simulink model "cable_driven_parallel_robot2022"  (R2022b)
settings: Solver=ode3  StartTime=0.0  StopTime=100  FixedStep=0.01  RelTol=1e-3
values from neighbouring files (symbols this model uses):
  cable_length = 1.2    [Model_Info.m]
  g = 9.81    [Model_Info.m]
  MP_H = 2    [Model_Info.m]
  MP_init_X = 0    [Model_Info.m]
  MP_init_Y = 0    [Model_Info.m]
  MP_init_Z = cable_length + (MP_H/2)    (= 2.2)    [Model_Info.m]
  MP_Ix = (MP_m/12)*(MP_W^2+MP_H^2)    (= 6.66666666667e-05)    [Model_Info.m]
  MP_Iy = (MP_m/12)*(MP_L^2+MP_H^2)    (= 6.66666666667e-05)    [Model_Info.m]
  MP_Iz = (MP_m/12)*(MP_L^2+MP_W^2)    (= 6.66666666667e-05)    [Model_Info.m]
  MP_L = 2    [Model_Info.m]
  MP_m = 0.0001    [Model_Info.m]
  MP_W = 2    [Model_Info.m]
  MR_init_X_L1 = -(MP_L/2)    (= -1)    [Model_Info.m]
  MR_init_X_L2 = (MP_L/2)    (= 1)    [Model_Info.m]
  MR_init_X_L3 = (MP_L/2)    (= 1)    [Model_Info.m]
  MR_init_X_L4 = -(MP_L/2)    (= -1)    [Model_Info.m]
  MR_init_Y_L1 = -(MP_W/2)    (= -1)    [Model_Info.m]
  MR_init_Y_L2 = -(MP_W/2)    (= -1)    [Model_Info.m]
  MR_init_Y_L3 = (MP_W/2)    (= 1)    [Model_Info.m]
  MR_init_Y_L4 = (MP_W/2)    (= 1)    [Model_Info.m]
  MR_init_Yaw_L1 = pi    (= 3.14159265359)    [Model_Info.m]
  MR_init_Yaw_L2 = 0    [Model_Info.m]
  MR_init_Yaw_L3 = 0    [Model_Info.m]
  MR_init_Yaw_L4 = pi    (= 3.14159265359)    [Model_Info.m]
  MR_Jr = (MR_m/12)*(MR_L^2+MR_W^2)    (= 0.333333333333)    [Model_Info.m]
  MR_m = 0.5    [Model_Info.m]
  MR_r = 2    [Model_Info.m]
  MR_WT = 2    [Model_Info.m]
  QR_Ax = 0.25*0    (= 0)    [Model_Info.m]
  QR_Ay = 0.25*0    (= 0)    [Model_Info.m]
  QR_Az = 0.25*0    (= 0)    [Model_Info.m]
  QR_b = 1.14*1e-7    (= 1.14e-07)    [Model_Info.m]
  QR_Ixx = 4.856*1e-3    (= 0.004856)    [Model_Info.m]
  QR_Iyy = 4.856*1e-3    (= 0.004856)    [Model_Info.m]
  QR_Izz = 8.801*1e-3    (= 0.008801)    [Model_Info.m]
  QR_K = 2.980*1e-6    (= 2.98e-06)    [Model_Info.m]
  QR_l = 0.225    [Model_Info.m]
  QR_m = 0.468    [Model_Info.m]
  QR_x0_U1 = -(MP_L/2)    (= -1)    [Model_Info.m]
  QR_x0_U2 = (MP_L/2)    (= 1)    [Model_Info.m]
  QR_x0_U3 = (MP_L/2)    (= 1)    [Model_Info.m]
  QR_x0_U4 = -(MP_L/2)    (= -1)    [Model_Info.m]
  QR_y0_U1 = -(MP_W/2)    (= -1)    [Model_Info.m]
  QR_y0_U2 = -(MP_W/2)    (= -1)    [Model_Info.m]
  QR_y0_U3 = (MP_W/2)    (= 1)    [Model_Info.m]
  QR_y0_U4 = (MP_W/2)    (= 1)    [Model_Info.m]
  QR_z0_U1 = 2*cable_length+(MP_H)    (= 4.4)    [Model_Info.m]
  QR_z0_U2 = 2*cable_length+(MP_H)    (= 4.4)    [Model_Info.m]
  QR_z0_U3 = 2*cable_length+(MP_H)    (= 4.4)    [Model_Info.m]
  QR_z0_U4 = 2*cable_length+(MP_H)    (= 4.4)    [Model_Info.m]
(part 5 of 12)

== system cable_driven_parallel_robot2022/Actuators-CableTension-MovingPlatform/QuadRotor1/Subsystem/Subsystem ==
  rest : Inport
  init : Inport  Port=2
  MATLAB Function : MATLAB Function  TreatAsAtomicUnit=on
  A_rest : Outport
  A_init : Outport  Port=2
  wires:
  MATLAB Function/2(init) -> A_init/1
  init/1 -> MATLAB Function/2(init0)
  MATLAB Function/1(rest) -> A_rest/1
  rest/1 -> MATLAB Function/1(rest0)

== system cable_driven_parallel_robot2022/Actuators-CableTension-MovingPlatform/QuadRotor1/Subsystem/Subsystem1 ==
  rest : Inport
  init : Inport  Port=2
  MATLAB Function : MATLAB Function  TreatAsAtomicUnit=on
  A_rest : Outport
  A_init : Outport  Port=2
  wires:
  MATLAB Function/2(init) -> A_init/1
  init/1 -> MATLAB Function/2(init0)
  MATLAB Function/1(rest) -> A_rest/1
  rest/1 -> MATLAB Function/1(rest0)

== system cable_driven_parallel_robot2022/Actuators-CableTension-MovingPlatform/QuadRotor1/Subsystem/Vel_Manager ==
  Demux : Demux  Outputs=3
  Demux1 : Demux  Outputs=8
  Terminator{,1..6} (7 alike) : Terminator
  Vx_min : Outport
  Vy_min : Outport  Port=2
  Vz_min : Outport  Port=3
  Reste : Outport  Port=4
  wires:
  Demux1/7 -> Terminator5/1
  Demux1/3 -> Terminator1/1
  [Vmin] -> Demux/1
  Demux1/8 -> Terminator6/1
  [isTension] -> Demux1/1
  Demux1/6 -> Terminator4/1
  Demux1/5 -> Terminator3/1
  Demux1/4 -> Terminator2/1
  Demux/1 -> Vx_min/1
  Demux/2 -> Vy_min/1
  Demux/3 -> Vz_min/1
  Demux1/2 -> Reste/1
  Demux1/1 -> Terminator/1

== system cable_driven_parallel_robot2022/Actuators-CableTension-MovingPlatform/QuadRotor2/Subsystem/Subsystem ==
  rest : Inport
  init : Inport  Port=2
  MATLAB Function : MATLAB Function  TreatAsAtomicUnit=on
  A_rest : Outport
  A_init : Outport  Port=2
  wires:
  rest/1 -> MATLAB Function/1(rest0)
  MATLAB Function/1(rest) -> A_rest/1
  init/1 -> MATLAB Function/2(init0)
  MATLAB Function/2(init) -> A_init/1

== system cable_driven_parallel_robot2022/Actuators-CableTension-MovingPlatform/QuadRotor2/Subsystem/Subsystem1 ==
  rest : Inport
  init : Inport  Port=2
  MATLAB Function : MATLAB Function  TreatAsAtomicUnit=on
  A_rest : Outport
  A_init : Outport  Port=2
  wires:
  rest/1 -> MATLAB Function/1(rest0)
  MATLAB Function/1(rest) -> A_rest/1
  init/1 -> MATLAB Function/2(init0)
  MATLAB Function/2(init) -> A_init/1

== system cable_driven_parallel_robot2022/Actuators-CableTension-MovingPlatform/QuadRotor2/Subsystem/Vel_Manager ==
  Demux : Demux  Outputs=3
  Demux1 : Demux  Outputs=8
  Terminator{,1..6} (7 alike) : Terminator
  Vx_min : Outport
  Vy_min : Outport  Port=2
  Vz_min : Outport  Port=3
  Reste : Outport  Port=4
  wires:
  Demux1/7 -> Terminator5/1
  [Vmin] -> Demux/1
  Demux1/8 -> Terminator6/1
  [isTension] -> Demux1/1
  Demux1/6 -> Terminator4/1
  Demux1/2 -> Terminator/1
  Demux1/5 -> Terminator3/1
  Demux1/4 -> Terminator2/1
  Demux/1 -> Vx_min/1
  Demux/2 -> Vy_min/1
  Demux/3 -> Vz_min/1
  Demux1/3 -> Reste/1
  Demux1/1 -> Terminator1/1

== system cable_driven_parallel_robot2022/Actuators-CableTension-MovingPlatform/QuadRotor3/Subsystem/Subsystem ==
  rest : Inport
  init : Inport  Port=2
  MATLAB Function : MATLAB Function  TreatAsAtomicUnit=on
  A_rest : Outport
  A_init : Outport  Port=2
  wires:
  MATLAB Function/2(init) -> A_init/1
  init/1 -> MATLAB Function/2(init0)
  MATLAB Function/1(rest) -> A_rest/1
  rest/1 -> MATLAB Function/1(rest0)

== system cable_driven_parallel_robot2022/Actuators-CableTension-MovingPlatform/QuadRotor3/Subsystem/Subsystem1 ==
  rest : Inport
  init : Inport  Port=2
  MATLAB Function : MATLAB Function  TreatAsAtomicUnit=on
  A_rest : Outport
  A_init : Outport  Port=2
  wires:
  MATLAB Function/2(init) -> A_init/1
  init/1 -> MATLAB Function/2(init0)
  MATLAB Function/1(rest) -> A_rest/1
  rest/1 -> MATLAB Function/1(rest0)

== system cable_driven_parallel_robot2022/Actuators-CableTension-MovingPlatform/QuadRotor3/Subsystem/Vel_Manager ==
  Demux : Demux  Outputs=3
  Demux1 : Demux  Outputs=8
  Terminator{,1..6} (7 alike) : Terminator
  Vx_min : Outport
  Vy_min : Outport  Port=2
  Vz_min : Outport  Port=3
  Reste : Outport  Port=4
  wires:
  Demux1/7 -> Terminator5/1
  Demux1/3 -> Terminator1/1
  [Vmin] -> Demux/1
  Demux1/8 -> Terminator6/1
  [isTension] -> Demux1/1
  Demux1/6 -> Terminator4/1
  Demux1/2 -> Terminator/1
  Demux1/5 -> Terminator3/1
  Demux/1 -> Vx_min/1
  Demux/2 -> Vy_min/1
  Demux/3 -> Vz_min/1
  Demux1/4 -> Reste/1
  Demux1/1 -> Terminator2/1

== matlab function cable_driven_parallel_robot2022/Target Wrench-Jacobian matrix/Subsystem/MATLAB Function4 ==
  data: T input; T_MP output; MP_Pose input; ME_Pose input; T_ME output
function [T_MP,T_ME] = fcn(T,MP_Pose,ME_Pose)

T_MP = zeros(3,1);

T_MP(1) = ((ME_Pose(1)-MP_Pose(1))/abs(ME_Pose(1)-MP_Pose(1)))*T(1);
T_MP(2) = ((ME_Pose(2)-MP_Pose(2))/abs(ME_Pose(2)-MP_Pose(2)))*T(2);
T_MP(3) = ((ME_Pose(3)-MP_Pose(3))/abs(ME_Pose(3)-MP_Pose(3)))*T(3);

T_ME = zeros(3,1);
T_ME(1) = ((MP_Pose(1)-ME_Pose(1))/abs(MP_Pose(1)-ME_Pose(1)))*T(1);
T_ME(2) = ((MP_Pose(2)-ME_Pose(2))/abs(MP_Pose(2)-ME_Pose(2)))*T(2);
T_ME(3) = ((MP_Pose(3)-ME_Pose(3))/abs(MP_Pose(3)-ME_Pose(3)))*T(3);

if( (ME_Pose(1)-MP_Pose(1)) == 0 )
    T_MP(1)=0;
    T_ME(1)=0;
end

if( (ME_Pose(2)-MP_Pose(2)) == 0 )
    T_MP(2)=0;
    T_ME(2)=0;
end

if( (ME_Pose(3)-MP_Pose(3)) == 0 )
    T_MP(3)=0;
    T_ME(3)=0;
end

== matlab function cable_driven_parallel_robot2022/Target Wrench-Jacobian matrix/Subsystem/MATLAB Function5 ==
  data: T input; T_MP output; MP_Pose input; ME_Pose input; T_ME output
function [T_MP,T_ME] = fcn(T,MP_Pose,ME_Pose)

T_MP = zeros(3,1);

T_MP(1) = ((ME_Pose(1)-MP_Pose(1))/abs(ME_Pose(1)-MP_Pose(1)))*T(1);
T_MP(2) = ((ME_Pose(2)-MP_Pose(2))/abs(ME_Pose(2)-MP_Pose(2)))*T(2);
T_MP(3) = ((ME_Pose(3)-MP_Pose(3))/abs(ME_Pose(3)-MP_Pose(3)))*T(3);

T_ME = zeros(3,1);
T_ME(1) = ((MP_Pose(1)-ME_Pose(1))/abs(MP_Pose(1)-ME_Pose(1)))*T(1);
T_ME(2) = ((MP_Pose(2)-ME_Pose(2))/abs(MP_Pose(2)-ME_Pose(2)))*T(2);
T_ME(3) = ((MP_Pose(3)-ME_Pose(3))/abs(MP_Pose(3)-ME_Pose(3)))*T(3);

if( (ME_Pose(1)-MP_Pose(1)) == 0 )
    T_MP(1)=0;
    T_ME(1)=0;
end

if( (ME_Pose(2)-MP_Pose(2)) == 0 )
    T_MP(2)=0;
    T_ME(2)=0;
end

if( (ME_Pose(3)-MP_Pose(3)) == 0 )
    T_MP(3)=0;
    T_ME(3)=0;
end

== matlab function cable_driven_parallel_robot2022/Target Wrench-Jacobian matrix/Subsystem/MATLAB Function6 ==
  data: T input; T_MP output; MP_Pose input; ME_Pose input; T_ME output
function [T_MP,T_ME] = fcn(T,MP_Pose,ME_Pose)

T_MP = zeros(3,1);

T_MP(1) = ((ME_Pose(1)-MP_Pose(1))/abs(ME_Pose(1)-MP_Pose(1)))*T(1);
T_MP(2) = ((ME_Pose(2)-MP_Pose(2))/abs(ME_Pose(2)-MP_Pose(2)))*T(2);
T_MP(3) = ((ME_Pose(3)-MP_Pose(3))/abs(ME_Pose(3)-MP_Pose(3)))*T(3);

T_ME = zeros(3,1);
T_ME(1) = ((MP_Pose(1)-ME_Pose(1))/abs(MP_Pose(1)-ME_Pose(1)))*T(1);
T_ME(2) = ((MP_Pose(2)-ME_Pose(2))/abs(MP_Pose(2)-ME_Pose(2)))*T(2);
T_ME(3) = ((MP_Pose(3)-ME_Pose(3))/abs(MP_Pose(3)-ME_Pose(3)))*T(3);

if( (ME_Pose(1)-MP_Pose(1)) == 0 )
    T_MP(1)=0;
    T_ME(1)=0;
end

if( (ME_Pose(2)-MP_Pose(2)) == 0 )
    T_MP(2)=0;
    T_ME(2)=0;
end

if( (ME_Pose(3)-MP_Pose(3)) == 0 )
    T_MP(3)=0;
    T_ME(3)=0;
end

== matlab function cable_driven_parallel_robot2022/Target Wrench-Jacobian matrix/Subsystem/MATLAB Function7 ==
  data: T input; T_MP output; MP_Pose input; ME_Pose input; T_ME output
function [T_MP,T_ME] = fcn(T,MP_Pose,ME_Pose)

T_MP = zeros(3,1);

T_MP(1) = ((ME_Pose(1)-MP_Pose(1))/abs(ME_Pose(1)-MP_Pose(1)))*T(1);
T_MP(2) = ((ME_Pose(2)-MP_Pose(2))/abs(ME_Pose(2)-MP_Pose(2)))*T(2);
T_MP(3) = ((ME_Pose(3)-MP_Pose(3))/abs(ME_Pose(3)-MP_Pose(3)))*T(3);

T_ME = zeros(3,1);
T_ME(1) = ((MP_Pose(1)-ME_Pose(1))/abs(MP_Pose(1)-ME_Pose(1)))*T(1);
T_ME(2) = ((MP_Pose(2)-ME_Pose(2))/abs(MP_Pose(2)-ME_Pose(2)))*T(2);
T_ME(3) = ((MP_Pose(3)-ME_Pose(3))/abs(MP_Pose(3)-ME_Pose(3)))*T(3);

if( (ME_Pose(1)-MP_Pose(1)) == 0 )
    T_MP(1)=0;
    T_ME(1)=0;
end

if( (ME_Pose(2)-MP_Pose(2)) == 0 )
    T_MP(2)=0;
    T_ME(2)=0;
end

if( (ME_Pose(3)-MP_Pose(3)) == 0 )
    T_MP(3)=0;
    T_ME(3)=0;
end

== matlab function cable_driven_parallel_robot2022/Target Wrench-Jacobian matrix/Subsystem/MATLAB Function8 ==
  data: T input; T_MP output; MP_Pose input; ME_Pose input; T_ME output
function [T_MP,T_ME] = fcn(T,MP_Pose,ME_Pose)

T_MP = zeros(3,1);

T_MP(1) = ((ME_Pose(1)-MP_Pose(1))/abs(ME_Pose(1)-MP_Pose(1)))*T(1);
T_MP(2) = ((ME_Pose(2)-MP_Pose(2))/abs(ME_Pose(2)-MP_Pose(2)))*T(2);
T_MP(3) = ((ME_Pose(3)-MP_Pose(3))/abs(ME_Pose(3)-MP_Pose(3)))*T(3);

T_ME = zeros(3,1);
T_ME(1) = ((MP_Pose(1)-ME_Pose(1))/abs(MP_Pose(1)-ME_Pose(1)))*T(1);
T_ME(2) = ((MP_Pose(2)-ME_Pose(2))/abs(MP_Pose(2)-ME_Pose(2)))*T(2);
T_ME(3) = ((MP_Pose(3)-ME_Pose(3))/abs(MP_Pose(3)-ME_Pose(3)))*T(3);

if( (ME_Pose(1)-MP_Pose(1)) == 0 )
    T_MP(1)=0;
    T_ME(1)=0;
end

if( (ME_Pose(2)-MP_Pose(2)) == 0 )
    T_MP(2)=0;
    T_ME(2)=0;
end

if( (ME_Pose(3)-MP_Pose(3)) == 0 )
    T_MP(3)=0;
    T_ME(3)=0;
end

== matlab function cable_driven_parallel_robot2022/Target Wrench-Jacobian matrix/Subsystem/MATLAB Function9 ==
  data: T input; T_MP output; MP_Pose input; ME_Pose input; T_ME output
function [T_MP,T_ME] = fcn(T,MP_Pose,ME_Pose)

T_MP = zeros(3,1);

T_MP(1) = ((ME_Pose(1)-MP_Pose(1))/abs(ME_Pose(1)-MP_Pose(1)))*T(1);
T_MP(2) = ((ME_Pose(2)-MP_Pose(2))/abs(ME_Pose(2)-MP_Pose(2)))*T(2);
T_MP(3) = ((ME_Pose(3)-MP_Pose(3))/abs(ME_Pose(3)-MP_Pose(3)))*T(3);

T_ME = zeros(3,1);
T_ME(1) = ((MP_Pose(1)-ME_Pose(1))/abs(MP_Pose(1)-ME_Pose(1)))*T(1);
T_ME(2) = ((MP_Pose(2)-ME_Pose(2))/abs(MP_Pose(2)-ME_Pose(2)))*T(2);
T_ME(3) = ((MP_Pose(3)-ME_Pose(3))/abs(MP_Pose(3)-ME_Pose(3)))*T(3);

if( (ME_Pose(1)-MP_Pose(1)) == 0 )
    T_MP(1)=0;
    T_ME(1)=0;
end

if( (ME_Pose(2)-MP_Pose(2)) == 0 )
    T_MP(2)=0;
    T_ME(2)=0;
end

if( (ME_Pose(3)-MP_Pose(3)) == 0 )
    T_MP(3)=0;
    T_ME(3)=0;
end

== matlab function cable_driven_parallel_robot2022/Target Wrench-Jacobian matrix/Subsystem/MATLAB Function10 ==
  data: T input; T_MP output; MP_Pose input; ME_Pose input; T_ME output
function [T_MP,T_ME] = fcn(T,MP_Pose,ME_Pose)

T_MP = zeros(3,1);

T_MP(1) = ((ME_Pose(1)-MP_Pose(1))/abs(ME_Pose(1)-MP_Pose(1)))*T(1);
T_MP(2) = ((ME_Pose(2)-MP_Pose(2))/abs(ME_Pose(2)-MP_Pose(2)))*T(2);
T_MP(3) = ((ME_Pose(3)-MP_Pose(3))/abs(ME_Pose(3)-MP_Pose(3)))*T(3);

T_ME = zeros(3,1);
T_ME(1) = ((MP_Pose(1)-ME_Pose(1))/abs(MP_Pose(1)-ME_Pose(1)))*T(1);
T_ME(2) = ((MP_Pose(2)-ME_Pose(2))/abs(MP_Pose(2)-ME_Pose(2)))*T(2);
T_ME(3) = ((MP_Pose(3)-ME_Pose(3))/abs(MP_Pose(3)-ME_Pose(3)))*T(3);

if( (ME_Pose(1)-MP_Pose(1)) == 0 )
    T_MP(1)=0;
    T_ME(1)=0;
end

if( (ME_Pose(2)-MP_Pose(2)) == 0 )
    T_MP(2)=0;
    T_ME(2)=0;
end

if( (ME_Pose(3)-MP_Pose(3)) == 0 )
    T_MP(3)=0;
    T_ME(3)=0;
end

== matlab function cable_driven_parallel_robot2022/Actuators-CableTension-MovingPlatform/Moving Platform/MATLAB Function ==
  data: T_Global input; roll input; pitch input; Tx_R output; yaw input; Ty_R output; Tz_R output
function [Tx_R,Ty_R,Tz_R] = fcn(T_Global,roll,pitch,yaw)

R_x = [1    0       0; ...
       0  cos(roll) -sin(roll); ...
       0  sin(roll) cos(roll)];
   
R_y = [cos(pitch)  0   sin(pitch); ...
       0           1         0; ...
      -sin(pitch) 0   cos(pitch)]; 
   
R_z = [cos(yaw) -sin(yaw)  0; ...
       sin(yaw)  cos(yaw)  0; ...
       0           0       1]; 

R = R_z*R_y*R_x;


TG=[T_Global(1);T_Global(2);T_Global(3)];



TR=R'*TG;

Tx_R = TR(1);
Ty_R = TR(2);
Tz_R = TR(3);

== matlab function cable_driven_parallel_robot2022/Actuators-CableTension-MovingPlatform/Moving Platform/MATLAB Function1 ==
  data: T_Global input; roll input; pitch input; Tx_R output; yaw input; Ty_R output; Tz_R output
function [Tx_R,Ty_R,Tz_R] = fcn(T_Global,roll,pitch,yaw)

R_x = [1    0       0; ...
       0  cos(roll) -sin(roll); ...
       0  sin(roll) cos(roll)];
   
R_y = [cos(pitch)  0   sin(pitch); ...
       0           1         0; ...
      -sin(pitch) 0   cos(pitch)]; 
   
R_z = [cos(yaw) -sin(yaw)  0; ...
       sin(yaw)  cos(yaw)  0; ...
       0           0       1]; 

R = R_z*R_y*R_x;


TG=[T_Global(1);T_Global(2);T_Global(3)];



TR=R'*TG;

Tx_R = TR(1);
Ty_R = TR(2);
Tz_R = TR(3);

== matlab function cable_driven_parallel_robot2022/Actuators-CableTension-MovingPlatform/Moving Platform/MATLAB Function2 ==
  data: T_Global input; roll input; pitch input; Tx_R output; yaw input; Ty_R output; Tz_R output
function [Tx_R,Ty_R,Tz_R] = fcn(T_Global,roll,pitch,yaw)

R_x = [1    0       0; ...
       0  cos(roll) -sin(roll); ...
       0  sin(roll) cos(roll)];
   
R_y = [cos(pitch)  0   sin(pitch); ...
       0           1         0; ...
      -sin(pitch) 0   cos(pitch)]; 
   
R_z = [cos(yaw) -sin(yaw)  0; ...
       sin(yaw)  cos(yaw)  0; ...
       0           0       1]; 

R = R_z*R_y*R_x;


TG=[T_Global(1);T_Global(2);T_Global(3)];



TR=R'*TG;

Tx_R = TR(1);
Ty_R = TR(2);
Tz_R = TR(3);

== matlab function cable_driven_parallel_robot2022/Actuators-CableTension-MovingPlatform/Moving Platform/MATLAB Function3 ==
  data: T_Global input; roll input; pitch input; Tx_R output; yaw input; Ty_R output; Tz_R output
function [Tx_R,Ty_R,Tz_R] = fcn(T_Global,roll,pitch,yaw)

R_x = [1    0       0; ...
       0  cos(roll) -sin(roll); ...
       0  sin(roll) cos(roll)];
   
R_y = [cos(pitch)  0   sin(pitch); ...
       0           1         0; ...
      -sin(pitch) 0   cos(pitch)]; 
   
R_z = [cos(yaw) -sin(yaw)  0; ...
       sin(yaw)  cos(yaw)  0; ...
       0           0       1]; 

R = R_z*R_y*R_x;


TG=[T_Global(1);T_Global(2);T_Global(3)];



TR=R'*TG;

Tx_R = TR(1);
Ty_R = TR(2);
Tz_R = TR(3);

== matlab function cable_driven_parallel_robot2022/Actuators-CableTension-MovingPlatform/Moving Platform/MATLAB Function4 ==
  data: T_Global input; roll input; pitch input; Tx_R output; yaw input; Ty_R output; Tz_R output
function [Tx_R,Ty_R,Tz_R] = fcn(T_Global,roll,pitch,yaw)

R_x = [1    0       0; ...
       0  cos(roll) -sin(roll); ...
       0  sin(roll) cos(roll)];
   
R_y = [cos(pitch)  0   sin(pitch); ...
       0           1         0; ...
      -sin(pitch) 0   cos(pitch)]; 
   
R_z = [cos(yaw) -sin(yaw)  0; ...
       sin(yaw)  cos(yaw)  0; ...
       0           0       1]; 

R = R_z*R_y*R_x;


TG=[T_Global(1);T_Global(2);T_Global(3)];



TR=R'*TG;

Tx_R = TR(1);
Ty_R = TR(2);
Tz_R = TR(3);

== matlab function cable_driven_parallel_robot2022/Actuators-CableTension-MovingPlatform/Moving Platform/MATLAB Function5 ==
  data: T_Global input; roll input; pitch input; Tx_R output; yaw input; Ty_R output; Tz_R output
function [Tx_R,Ty_R,Tz_R] = fcn(T_Global,roll,pitch,yaw)

R_x = [1    0       0; ...
       0  cos(roll) -sin(roll); ...
       0  sin(roll) cos(roll)];
   
R_y = [cos(pitch)  0   sin(pitch); ...
       0           1         0; ...
      -sin(pitch) 0   cos(pitch)]; 
   
R_z = [cos(yaw) -sin(yaw)  0; ...
       sin(yaw)  cos(yaw)  0; ...
       0           0       1]; 

R = R_z*R_y*R_x;


TG=[T_Global(1);T_Global(2);T_Global(3)];



TR=R'*TG;

Tx_R = TR(1);
Ty_R = TR(2);
Tz_R = TR(3);

== matlab function cable_driven_parallel_robot2022/Actuators-CableTension-MovingPlatform/Moving Platform/MATLAB Function6 ==
  data: T_Global input; roll input; pitch input; Tx_R output; yaw input; Ty_R output; Tz_R output
function [Tx_R,Ty_R,Tz_R] = fcn(T_Global,roll,pitch,yaw)

R_x = [1    0       0; ...
       0  cos(roll) -sin(roll); ...
       0  sin(roll) cos(roll)];
   
R_y = [cos(pitch)  0   sin(pitch); ...
       0           1         0; ...
      -sin(pitch) 0   cos(pitch)]; 
   
R_z = [cos(yaw) -sin(yaw)  0; ...
       sin(yaw)  cos(yaw)  0; ...
       0           0       1]; 

R = R_z*R_y*R_x;


TG=[T_Global(1);T_Global(2);T_Global(3)];



TR=R'*TG;

Tx_R = TR(1);
Ty_R = TR(2);
Tz_R = TR(3);

== matlab function cable_driven_parallel_robot2022/Actuators-CableTension-MovingPlatform/2 Wheels Diffrential Mobile Robot/2 Wheels Diffrential Mobile Robot/2 Wheels Diffrential Mobile Robot Transformation to Global ==
  settings: updateMethod=DISCRETE
  data: Vx input; Vy input; Vz input; yaw input; Vbx output; Vby output; Vbz output; Vx_min input; Vy_min input; Vz_min input; reste input; z input; rest output
function [Vbx,Vby,Vbz,rest] = fcn(Vx,Vy,Vz,yaw,Vx_min,Vy_min,Vz_min,reste,z)
rest=0;
a=[Vx;Vy;Vz];

R_z = [cos(yaw) -sin(yaw)  0; ...
       sin(yaw)  cos(yaw)  0; ...
       0           0       1]; 

Vel=R_z*a;

Vbx = Vel(1);

Vby = Vel(2);

Vbz = Vel(3);

if reste ==1
    Vbx = Vx_min;

    Vby = Vy_min;

    Vbz = Vz_min;
end

if ((Vbz<0 && z ==0) || z<0)
    rest=1;
    Vbz=0;    
end

== matlab function cable_driven_parallel_robot2022/Actuators-CableTension-MovingPlatform/Moving Platform/MATLAB Function7 ==
  data: T_Global input; roll input; pitch input; Tx_R output; yaw input; Ty_R output; Tz_R output
function [Tx_R,Ty_R,Tz_R] = fcn(T_Global,roll,pitch,yaw)

R_x = [1    0       0; ...
       0  cos(roll) -sin(roll); ...
       0  sin(roll) cos(roll)];
   
R_y = [cos(pitch)  0   sin(pitch); ...
       0           1         0; ...
      -sin(pitch) 0   cos(pitch)]; 
   
R_z = [cos(yaw) -sin(yaw)  0; ...
       sin(yaw)  cos(yaw)  0; ...
       0           0       1]; 

R = R_z*R_y*R_x;


TG=[T_Global(1);T_Global(2);T_Global(3)];



TR=R'*TG;

Tx_R = TR(1);
Ty_R = TR(2);
Tz_R = TR(3);

== matlab function cable_driven_parallel_robot2022/Actuators-CableTension-MovingPlatform/2 Wheels Diffrential Mobile Robot/MATLAB Function7 ==
  data: T_Global input; roll input; pitch input; Tx_R output; yaw input; Ty_R output; Tz_R output
function [Tx_R,Ty_R,Tz_R] = fcn(T_Global,roll,pitch,yaw)

R_x = [1    0       0; ...
       0  cos(roll) -sin(roll); ...
       0  sin(roll) cos(roll)];
   
R_y = [cos(pitch)  0   sin(pitch); ...
       0           1         0; ...
      -sin(pitch) 0   cos(pitch)]; 
   
R_z = [cos(yaw) -sin(yaw)  0; ...
       sin(yaw)  cos(yaw)  0; ...
       0           0       1]; 

R = R_z*R_y*R_x;


TG=[T_Global(1);T_Global(2);T_Global(3)];



TR=R'*TG;

Tx_R = TR(1);
Ty_R = TR(2);
Tz_R = TR(3);

== matlab function cable_driven_parallel_robot2022/Actuators-CableTension-MovingPlatform/2 Wheels Diffrential Mobile Robot1/2 Wheels Diffrential Mobile Robot/2 Wheels Diffrential Mobile Robot ==
  settings: updateMethod=DISCRETE
  data: TR input; TL input; Tx input; Ty input; Tz input; Jr input; mr input; r input; ax output; ay output; az output; alpha_r output; WT input
function [ax,ay,az,alpha_r] = fcn(TR,TL,Tx,Ty,Tz,Jr,mr,r,WT)


g=9.81;

ax = ((TR/r)+(TL/r)+Tx)/mr;
ay = (Ty)/mr;
az = (Tz -mr*g)/mr;


alpha_r = ((TR-TL)*(WT/2*r))/Jr;

== matlab function cable_driven_parallel_robot2022/Actuators-CableTension-MovingPlatform/2 Wheels Diffrential Mobile Robot1/2 Wheels Diffrential Mobile Robot/2 Wheels Diffrential Mobile Robot Transformation to Global ==
  settings: updateMethod=DISCRETE
  data: Vx input; Vy input; Vz input; yaw input; Vbx output; Vby output; Vbz output; Vx_min input; Vy_min input; Vz_min input; reste input; z input; rest output
function [Vbx,Vby,Vbz,rest] = fcn(Vx,Vy,Vz,yaw,Vx_min,Vy_min,Vz_min,reste,z)
rest=0;
a=[Vx;Vy;Vz];

R_z = [cos(yaw) -sin(yaw)  0; ...
       sin(yaw)  cos(yaw)  0; ...
       0           0       1]; 

Vel=R_z*a;

Vbx = Vel(1);

Vby = Vel(2);

Vbz = Vel(3);

if reste ==1
    Vbx = Vx_min;

    Vby = Vy_min;

    Vbz = Vz_min;
end

if ((Vbz<0 && z ==0) || z<0)
    rest=1;
    Vbz=0;    
end

== matlab function cable_driven_parallel_robot2022/Actuators-CableTension-MovingPlatform/2 Wheels Diffrential Mobile Robot1/MATLAB Function7 ==
  data: T_Global input; roll input; pitch input; Tx_R output; yaw input; Ty_R output; Tz_R output
function [Tx_R,Ty_R,Tz_R] = fcn(T_Global,roll,pitch,yaw)

R_x = [1    0       0; ...
       0  cos(roll) -sin(roll); ...
       0  sin(roll) cos(roll)];
   
R_y = [cos(pitch)  0   sin(pitch); ...
       0           1         0; ...
      -sin(pitch) 0   cos(pitch)]; 
   
R_z = [cos(yaw) -sin(yaw)  0; ...
       sin(yaw)  cos(yaw)  0; ...
       0           0       1]; 

R = R_z*R_y*R_x;


TG=[T_Global(1);T_Global(2);T_Global(3)];



TR=R'*TG;

Tx_R = TR(1);
Ty_R = TR(2);
Tz_R = TR(3);

== matlab function cable_driven_parallel_robot2022/Actuators-CableTension-MovingPlatform/2 Wheels Diffrential Mobile Robot2/2 Wheels Diffrential Mobile Robot/2 Wheels Diffrential Mobile Robot ==
  settings: updateMethod=DISCRETE
  data: TR input; TL input; Tx input; Ty input; Tz input; Jr input; mr input; r input; ax output; ay output; az output; alpha_r output; WT input
function [ax,ay,az,alpha_r] = fcn(TR,TL,Tx,Ty,Tz,Jr,mr,r,WT)


g=9.81;

ax = ((TR/r)+(TL/r)+Tx)/mr;
ay = (Ty)/mr;
az = (Tz -mr*g)/mr;

alpha_r = ((TR-TL)*(WT/2*r))/Jr;

== matlab function cable_driven_parallel_robot2022/Actuators-CableTension-MovingPlatform/2 Wheels Diffrential Mobile Robot2/2 Wheels Diffrential Mobile Robot/2 Wheels Diffrential Mobile Robot Transformation to Global ==
  settings: updateMethod=DISCRETE
  data: Vx input; Vy input; Vz input; yaw input; Vbx output; Vby output; Vbz output; Vx_min input; Vy_min input; Vz_min input; reste input; z input; rest output
function [Vbx,Vby,Vbz,rest] = fcn(Vx,Vy,Vz,yaw,Vx_min,Vy_min,Vz_min,reste,z)
rest=0;
a=[Vx;Vy;Vz];

R_z = [cos(yaw) -sin(yaw)  0; ...
       sin(yaw)  cos(yaw)  0; ...
       0           0       1]; 

Vel=R_z*a;

Vbx = Vel(1);

Vby = Vel(2);

Vbz = Vel(3);

if reste ==1
    Vbx = Vx_min;

    Vby = Vy_min;

    Vbz = Vz_min;
end

if ((Vbz<0 && z ==0) || z<0)
    rest=1;
    Vbz=0;    
end

== matlab function cable_driven_parallel_robot2022/Actuators-CableTension-MovingPlatform/2 Wheels Diffrential Mobile Robot2/MATLAB Function7 ==
  data: T_Global input; roll input; pitch input; Tx_R output; yaw input; Ty_R output; Tz_R output
function [Tx_R,Ty_R,Tz_R] = fcn(T_Global,roll,pitch,yaw)

R_x = [1    0       0; ...
       0  cos(roll) -sin(roll); ...
       0  sin(roll) cos(roll)];
   
R_y = [cos(pitch)  0   sin(pitch); ...
       0           1         0; ...
      -sin(pitch) 0   cos(pitch)]; 
   
R_z = [cos(yaw) -sin(yaw)  0; ...
       sin(yaw)  cos(yaw)  0; ...
       0           0       1]; 

R = R_z*R_y*R_x;


TG=[T_Global(1);T_Global(2);T_Global(3)];



TR=R'*TG;

Tx_R = TR(1);
Ty_R = TR(2);
Tz_R = TR(3);

== matlab function cable_driven_parallel_robot2022/Actuators-CableTension-MovingPlatform/2 Wheels Diffrential Mobile Robot3/2 Wheels Diffrential Mobile Robot/2 Wheels Diffrential Mobile Robot ==
  settings: updateMethod=DISCRETE
  data: TR input; TL input; Tx input; Ty input; Tz input; Jr input; mr input; r input; ax output; ay output; az output; alpha_r output; WT input
function [ax,ay,az,alpha_r] = fcn(TR,TL,Tx,Ty,Tz,Jr,mr,r,WT)

g=9.81;

ax = ((TR/r)+(TL/r)+Tx)/mr;
ay = (Ty)/mr;
az = (Tz -mr*g)/mr;

alpha_r = ((TR-TL)*(WT/2*r))/Jr;

== matlab function cable_driven_parallel_robot2022/Actuators-CableTension-MovingPlatform/2 Wheels Diffrential Mobile Robot3/2 Wheels Diffrential Mobile Robot/2 Wheels Diffrential Mobile Robot Transformation to Global ==
  settings: updateMethod=DISCRETE
  data: Vx input; Vy input; Vz input; yaw input; Vbx output; Vby output; Vbz output; Vx_min input; Vy_min input; Vz_min input; reste input; z input; rest output
function [Vbx,Vby,Vbz,rest] = fcn(Vx,Vy,Vz,yaw,Vx_min,Vy_min,Vz_min,reste,z)
rest=0;

a=[Vx;Vy;Vz];

R_z = [cos(yaw) -sin(yaw)  0; ...
       sin(yaw)  cos(yaw)  0; ...
       0           0       1]; 

Vel=R_z*a;

Vbx = Vel(1);

Vby = Vel(2);

Vbz = Vel(3);

if reste ==1
    Vbx = Vx_min;

    Vby = Vy_min;

    Vbz = Vz_min;
end

if ((Vbz<0 && z ==0) || z<0)
    rest=1;
    Vbz=0;    
end

== matlab function cable_driven_parallel_robot2022/Actuators-CableTension-MovingPlatform/2 Wheels Diffrential Mobile Robot3/MATLAB Function7 ==
  data: T_Global input; roll input; pitch input; Tx_R output; yaw input; Ty_R output; Tz_R output
function [Tx_R,Ty_R,Tz_R] = fcn(T_Global,roll,pitch,yaw)

R_x = [1    0       0; ...
       0  cos(roll) -sin(roll); ...
       0  sin(roll) cos(roll)];
   
R_y = [cos(pitch)  0   sin(pitch); ...
       0           1         0; ...
      -sin(pitch) 0   cos(pitch)]; 
   
R_z = [cos(yaw) -sin(yaw)  0; ...
       sin(yaw)  cos(yaw)  0; ...
       0           0       1]; 

R = R_z*R_y*R_x;


TG=[T_Global(1);T_Global(2);T_Global(3)];



TR=R'*TG;

Tx_R = TR(1);
Ty_R = TR(2);
Tz_R = TR(3);
